simulink model "T1_validacao_sinais"  (R2026a)
settings: Solver=FixedStepDiscrete  StopTime=0.03333282470703125  FixedStep=5.0862630208333333e-07
settings Model: Creator=vitor  LastModifiedBy=vitor

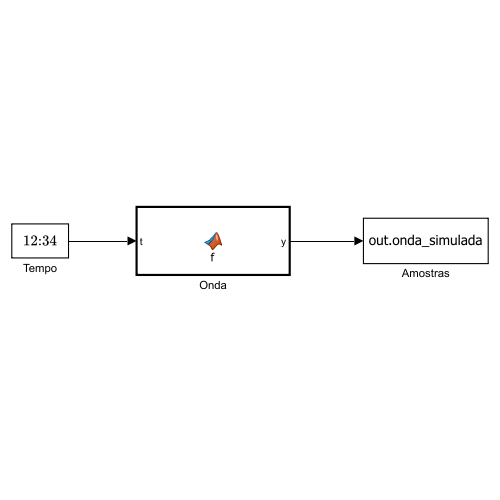
[thumbnail: Simulink's stored preview of the top-level diagram]
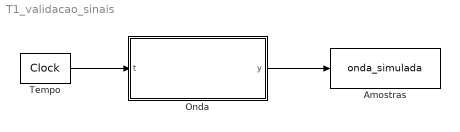
== system T1_validacao_sinais ==
  Amostras : ToWorkspace  VariableName=onda_simulada  SaveFormat=Timeseries  SampleTime=-1
  Onda : MATLAB Function  TreatAsAtomicUnit=on
  Tempo : DigitalClock  SampleTime=5.0862630208333333e-07
  wires:
  Tempo/1 -> Onda/1(t)
  Onda/1(y) -> Amostras/1

== matlab function T1_validacao_sinais/Onda ==
  data: t input; y output
function y = f(t)
x=376.99111843077515*(t+5.0862630208333333e-07/2);
A=1; L=12.566370614359172; phi=1.0471975511965976;
z=mod(x,L);
ligado=(z>=phi)&&(z<phi+2.0943951023931953);
ligado=ligado||((z>=7.8539816339744828)&&(z<10.995574287564276));
y=A*double(ligado);
y=2*y-A;
end
